simulink model "hopper_6dof_NED_v2_fluid_integration"  (R2026a)
settings: Solver=FixedStepAuto  StopTime=tgrid(end)  FixedStep=1e-3  RelTol=1e-5
InitFcn:
  | load('FuelPropsData.mat');
undefined symbols (not defined in the file): cg_init, dcg_dMfu_table, dcg_dMox_table, dI_dMfu_table, dI_dMox_table, ENGINE, engine_cg, engine_mass, fu_axial_damping_ratios, fu_lateral_damping_ratios, fu_mass_profile, fu_masses, fu_mdot_data, g, IN, K1flat, K2grid, MoI_init, mount_cg, OUT, ox_axial_damping_ratios, ox_lateral_damping_ratios, ox_mass_profile, ox_masses, ox_mdot_data, pressureLevels, r_leg, r_leg_1, r_leg_2, r_leg_3, r_leg_4, STRUCT, tank_r, TANKS, Target_Trajectory, tgrid, thrust_data, unom, uwndTable, VEH, vwndTable
libraries: fl_lib x43, nesl_utility x31, matrix_library x18, SimscapeFluids_lib x13, simulink x8, simulink_extras x7, slpidlib x7, dspindex x3, dspmtrx3 x3, sl_discontinuities x2, aerolibanim x1, commrandsrc3 x1
(part 1 of 7)
settings Model: Creator=asing  LastModifiedBy=asing
settings DebuggingCC: SignalInfNanChecking=warning
settings SimscapeCC: SimscapeNominalValues="[{\"value\":\"1\",\"unit\":\"A\"},{\"value\":\"1\",\"unit\":\"bar\"},{\"value\":\"1\",\"unit\":\"cm^2\"},{\"value\":\"1\",\"unit\":\"cm^3/s\"},{\"value\":\"1\",\"unit\":\"kJ/kg\"},{\"value\":\"1\",\"unit\":\"kW\"},{\"value\":\"1\",\"unit\":\"l\"},{\"value\":\"1\",\"unit\":\"N\"},{\"value\":\"1\",\"unit\":\"N*m\"},{\"value\":\"1\",\"unit\":\"V\"}]"  SimscapeLogType=none  SimscapeLogDataHistory=5000.0

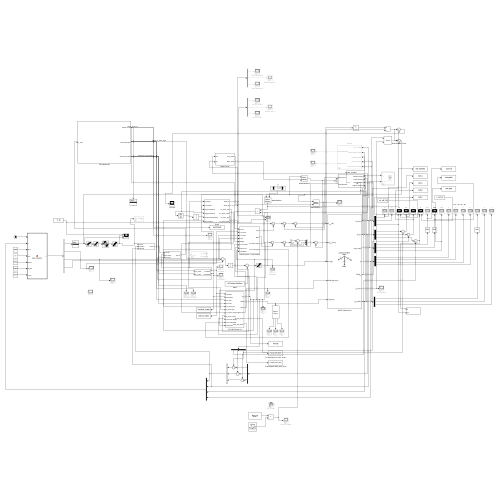
[thumbnail: Simulink's stored preview of the top-level diagram]
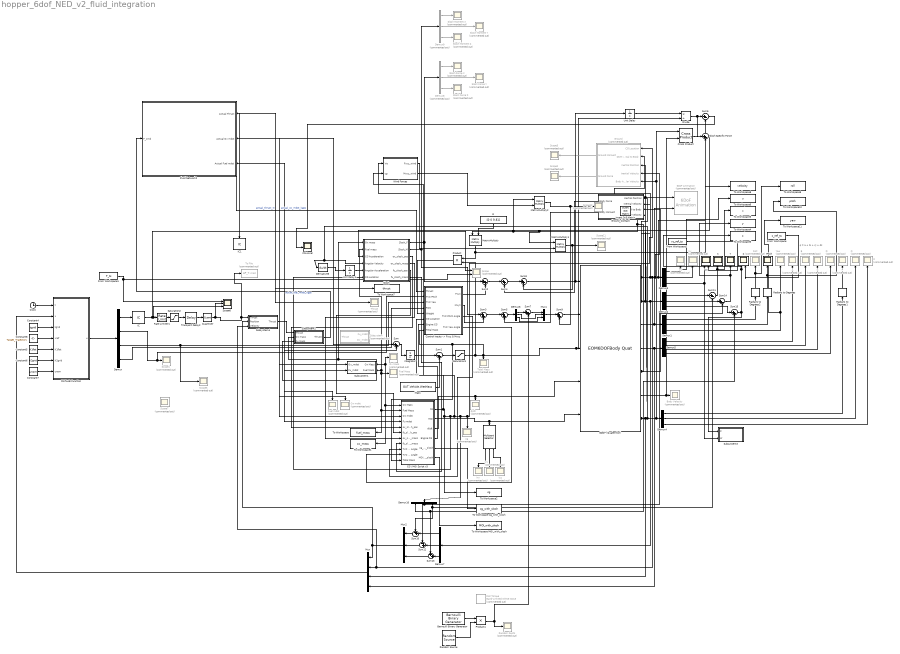
== system hopper_6dof_NED_v2_fluid_integration ==
  note: q = a + bi + cj + dk
  " " : dspindex/Multiport Selector  rowsOrCols=Rows  idxCellArray={1,2,3}  idxErrMode=Clip Index
      settings: LibrarySourceBlock=|
      | dsphdlsupportsigmgmt/Multiport
      | Selector
  6DOF (Quaternion) : EOM6DOFBodyQuat  mtype=Custom Variable  xme_0=[0 0 -cg_init]  eul_0=[0 pi/2 0]
  6DoF Animation : aerolibanim/6DoF Animation  Commented=on  u1=[0 200 -200 200 -100 5]  u2=0.1  u3=2  u4=[4000 0 -5000]  u5=Fly alongside  u6=[100 100 -50]  u7=10  u8=on
  A : Scope  Commented=on
      settings: ActiveDisplayYMinimum=-1  ActiveDisplayYMaximum=1  DataLoggingVariableName=ScopeData12
  B : Scope  Commented=on
      settings: ActiveDisplayYMinimum=-1  ActiveDisplayYMaximum=1  DataLoggingVariableName=ScopeData13
  Bernoulli Binary Generator : commrandsrc3/Bernoulli Binary Generator  ProbabilityOfZero=0.95  SeedSource=Parameter  Seed=0  SampleTime=0.1  SamplesPerFrame=1  OutputDataType=double  SimulateUsing=Interpreted execution
  Body Velocity : Scope  Commented=on
      settings: ActiveDisplayYMinimum=-9.910378836747423  ActiveDisplayYMaximum=88.214312640198585  DataLoggingVariableName=ScopeData29
  C : Scope  Commented=on
      settings: DataLoggingVariableName=ScopeData14
  CG / MOI Script v3 : Subsystem
  CG Accel : Scope
      settings: ActiveDisplayYMinimum=-11.407629776225166  ActiveDisplayYMaximum=3.5948297727236085  DataLoggingVariableName=ScopeData33
  Clock : Clock
  Constant4 : Constant  Value=tgrid
  Constant5 : Constant  Value=K1flat
  Constant6 : Constant  Value=K2grid
  Constant7 : Constant  Value=unom
  Constant8 : Constant  Value=Target_Trajectory
  "Control Inputs -> Fxyz & Mxyz" : Subsystem
  Cross Product : matrix_library/Cross Product
  D : Scope  Commented=on
      settings: DataLoggingVariableName=ScopeData15
  Demux : Demux
  Demux{1..4,6..7,10} (7 alike) : Demux  Outputs=3
  Demux5 : Demux
  Demux8 : Demux  Commented=on  Outputs=3
  Demux9 : Demux  Commented=on  Outputs=3
  Derivative3 : Derivative  CoefficientInTFapproximation=3
  Divide : Product  Inputs=*/
  Fluid Network2 : Subsystem
  From Workspace : FromWorkspace  VariableName=z_ref_ts
  From Workspace1 : FromWorkspace  VariableName=T_ts
  From Workspace2 : FromWorkspace  VariableName=vz_ref_ts
  Fuel Mass : Scope  Commented=on
      settings: ActiveDisplayYMinimum=7.5154679010584076  ActiveDisplayYMaximum=13.609392455437956  DataLoggingVariableName=ScopeData18
  Fuel mdot : Scope  Commented=on
      settings: ActiveDisplayYMinimum=-0.057229294241176995  ActiveDisplayYMaximum=0.515142758459371  DataLoggingVariableName=ScopeData20
  "Ground " : Subsystem  Commented=on
  Ground_Contact : Subsystem
  IC : InitialCondition  Value=VEH.mass.wet*g
  IC1 : InitialCondition  Value=VEH.mass.wet*g
  Integrator : Integrator
  Invert 3x3 Matrix : aerolibutil/Invert  3x3 Matrix
  Ixx : Scope  Commented=on
      settings: ActiveDisplayYMinimum=-1.2693672305907171  ActiveDisplayYMaximum=1.7662706804264152  DataLoggingVariableName=ScopeData21
  Iyy : Scope  Commented=on
      settings: ActiveDisplayYMinimum=-8.2381488489345962  ActiveDisplayYMaximum=64.485305245521346  DataLoggingVariableName=ScopeData26
  Izz : Scope  Commented=on
      settings: ActiveDisplayYMinimum=-8.2393172969859414  ActiveDisplayYMaximum=64.3796161087634  DataLoggingVariableName=ScopeData27
  MATLAB Function : MATLAB Function  TreatAsAtomicUnit=on
  Mass : Constant  Value=OUT.Vehicle.WetMass
  MatrixMultiply : Product  Multiplication=Matrix(*)
  MatrixMultiply1 : Product  Multiplication=Matrix(*)
  MatrixMultiply2 : Product  Multiplication=Matrix(*)
  Mux : Mux
  Mux1 : Mux  Inputs=3
  Mux2 : Mux  Inputs=3
  Ox Mass : Scope  Commented=on
      settings: ActiveDisplayYMinimum=9.14433500982005  ActiveDisplayYMaximum=16.761740554464438  DataLoggingVariableName=ScopeData17
  Ox mdot : Scope  Commented=on
      settings: ActiveDisplayYMinimum=-0.071536617800839461  ActiveDisplayYMaximum=0.64392844807434468  DataLoggingVariableName=ScopeData19
  P : Scope  Commented=on
      settings: ActiveDisplayYMinimum=-40.272034282628653  ActiveDisplayYMaximum=40.18271139614702  DataLoggingVariableName=ScopeData9
  Pitch : Scope
      settings: ActiveDisplayYMinimum=43.438097555335354  ActiveDisplayYMaximum=90.504604934017451  DataLoggingVariableName=ScopeData4
  Product : Product
  Product1 : Product
  Q : Scope  Commented=on
      settings: ActiveDisplayYMinimum=-0.03908687484475059  ActiveDisplayYMaximum=0.052615482319584864  DataLoggingVariableName=ScopeData10
  Quantizer : Quantizer  QuantizationInterval=IN.throttle_valve.resolution
  R : Scope  Commented=on
      settings: ActiveDisplayYMinimum=-0.0070860969112896514  ActiveDisplayYMaximum=0.0085398632976064828  DataLoggingVariableName=ScopeData11
  Radians to Degrees : simulink_extras/Transformations/Radians to Degrees
  Radians to Degrees1 : simulink_extras/Transformations/Radians to Degrees
  Radians to Degrees2 : simulink_extras/Transformations/Radians to Degrees
  Random Source : dspsrcs4/Random Source  SrcType=Gaussian  MinVal=0  MaxVal=1  MeanVal=0  VarVal=20  RepMode=Specify seed  rawSeed=1  IsInherit=off  SampTime=1  SampFrame=1  OutComplex=Real  DataType=double  SimulateUsing=Interpreted execution
  Random Gusts : Scope  Commented=on
      settings: ActiveDisplayYMinimum=-8.5897961122323956  ActiveDisplayYMaximum=9.8055336087823335  DataLoggingVariableName=ScopeData63
  Rate Limiter1 : RateLimiter  RisingSlewLimit=IN.throttle_valve.rate_limit  FallingSlewLimit=-IN.throttle_valve.rate_limit  SampleTimeMode=inherited
  Roll : Scope  Commented=on
      settings: ActiveDisplayYMinimum=-204.65947396986587  ActiveDisplayYMaximum=175.17097918939032  DataLoggingVariableName=ScopeData3
  Roll Torque : simulink/Sources/Band-Limited White Noise  Commented=on  Cov=5  Ts=1  seed=[23341]
  Saturation1 : Saturate  UpperLimit=OUT.Vehicle.WetMass  LowerLimit=OUT.Vehicle.DryMass
  Saturation2 : Saturate  UpperLimit=IN.propulsion.nominal_thrust * IN.propulsion.throttle_range(2)  LowerLimit=IN.propulsion.nominal_thrust * IN.propulsion.throttle_range(1)
  Scope : Scope  Commented=on  NumInputPorts=2
      settings: ActiveDisplayYMinimum=725.64918679567745  ActiveDisplayYMaximum=1423.3753088923004  DataLoggingVariableName=ScopeData52
  Scope{1..3,5,7,11..12} (7 alike) : Scope  Commented=on
      Scope1 settings: ActiveDisplayYMinimum=-0.00050229611394169284  ActiveDisplayYMaximum=0.0028458999197228797  DataLoggingVariableName=ScopeData53
      Scope11 settings: ActiveDisplayYMinimum=-1.725572479086533  ActiveDisplayYMaximum=0.1917302754540588  DataLoggingVariableName=ScopeData66
      Scope12 settings: ActiveDisplayYMinimum=-2.88543679656206  ActiveDisplayYMaximum=6.7910588943113428  DataLoggingVariableName=ScopeData67
      Scope2 settings: ActiveDisplayYMinimum=-8449.52436564975  ActiveDisplayYMaximum=76045.719290847759  DataLoggingVariableName=ScopeData49
      Scope3 settings: ActiveDisplayYMinimum=-903.54597657114152  ActiveDisplayYMaximum=89.720851920197276  DataLoggingVariableName=ScopeData51
      Scope5 settings: ActiveDisplayYMinimum=-0.0014807269526439936  ActiveDisplayYMaximum=0.00063209871075060983  DataLoggingVariableName=ScopeData57
      Scope7 settings: ActiveDisplayYMinimum=-9.3466701964128269  ActiveDisplayYMaximum=8.508922841651323  DataLoggingVariableName=ScopeData62
  Scope6 : Scope  NumInputPorts=3
      settings: ActiveDisplayYMinimum=-12632.794590273525  ActiveDisplayYMaximum=4410.2403285914115  DataLoggingVariableName=ScopeData59
  Slosh : Subsystem
  Slosh Force X : Scope  Commented=on
      settings: ActiveDisplayYMinimum=-23.703787957912279  ActiveDisplayYMaximum=30.843704332518367  DataLoggingVariableName=ScopeData32
  Slosh Force Y : Scope  Commented=on
      settings: ActiveDisplayYMinimum=-0.5552642189596475  ActiveDisplayYMaximum=0.52836332227705041  DataLoggingVariableName=ScopeData72
  Slosh Force Z : Scope  Commented=on
      settings: ActiveDisplayYMinimum=-0.4568274165323904  ActiveDisplayYMaximum=0.43197139726332079  DataLoggingVariableName=ScopeData73
  Slosh Moment X : Scope  Commented=on
      settings: ActiveDisplayYMinimum=-1  ActiveDisplayYMaximum=1  DataLoggingVariableName=ScopeData74
  Slosh Moment Y : Scope  Commented=on
      settings: ActiveDisplayYMinimum=-0.020821390947241118  ActiveDisplayYMaximum=0.019580844558623325  DataLoggingVariableName=ScopeData75
  Slosh Moment Z : Scope  Commented=on
      settings: ActiveDisplayYMinimum=-0.045380586631965543  ActiveDisplayYMaximum=0.048640802204673789  DataLoggingVariableName=ScopeData76
  Slosh Specific Force : Sum  Description=(F_total/m) - g_body = non-gravitational specific force at the CG; drives the slosh pendulums.  Inputs=|+-
  Subsystem : Subsystem  Commented=on
  Subsystem1 : Subsystem
  Subsystem2 : Subsystem
  Subsystem3 : Subsystem
  Subsystem4 : Subsystem
  Sum{,2..5,7..9,15} (9 alike) : Sum  Inputs=|++
  Sum1 : Sum  Inputs=|-+
  Sum10 : Sum  Inputs=-+|
  Sum11 : Sum  Inputs=|+-
  Sum12 : Sum  Inputs=-+|
  Sum13 : Sum  Inputs=++|
  Sum14 : Sum  Inputs=|+-
  Sum6 : Sum  Inputs=|+-
  Thrust : Scope  Commented=on
      settings: ActiveDisplayYMinimum=-212.49999999999994  ActiveDisplayYMaximum=1912.5  DataLoggingVariableName=ScopeData25
  To File : ToFile  Commented=on  Filename=AP_T.mat  SaveFormat=Timeseries
  To Workspace : ToWorkspace  VariableName=fuel_mass  SaveFormat=Timeseries  SampleTime=-1
  To Workspace MOI_with_slosh : ToWorkspace  VariableName=MOI_with_slosh  SaveFormat=Timeseries  SampleTime=-1
  To Workspace cg_with_slosh : ToWorkspace  VariableName=cg_with_slosh  SaveFormat=Timeseries  SampleTime=-1
  To Workspace1 : ToWorkspace  VariableName=ox_mass  SaveFormat=Timeseries  SampleTime=-1
  To Workspace10 : ToWorkspace  VariableName=pitch  SaveFormat=Timeseries  SampleTime=-1
  To Workspace11 : ToWorkspace  VariableName=yaw  SaveFormat=Timeseries  SampleTime=-1
  To Workspace2 : ToWorkspace  VariableName=cg  SaveFormat=Timeseries  SampleTime=-1
  To Workspace3 : ToWorkspace  VariableName=x  SaveFormat=Timeseries  SampleTime=-1
  To Workspace4 : ToWorkspace  VariableName=y  SaveFormat=Timeseries  SampleTime=-1
  To Workspace5 : ToWorkspace  VariableName=z  SaveFormat=Timeseries  SampleTime=-1
  To Workspace6 : ToWorkspace  VariableName=u  SaveFormat=Timeseries  SampleTime=-1
  To Workspace7 : ToWorkspace  VariableName=thrust  SaveFormat=Timeseries  SampleTime=-1
  To Workspace8 : ToWorkspace  VariableName=velocity  SaveFormat=Timeseries  SampleTime=-1
  To Workspace9 : ToWorkspace  VariableName=roll  SaveFormat=Timeseries  SampleTime=-1
  Total Mass : Scope  Commented=on
      settings: ActiveDisplayYMinimum=123.40007682459402  ActiveDisplayYMaximum=148.35554701948959  DataLoggingVariableName=ScopeData16
  Transport Delay2 : TransportDelay  DelayTime=IN.throttle_valve_latency
  Unit Delay : UnitDelay  SampleTime=-1
  Unit Delay1 : UnitDelay  SampleTime=-1
  Vx : Scope  Commented=on
      settings: ActiveDisplayYMinimum=-1.0568314607793221  ActiveDisplayYMaximum=0.63247821872235255  DataLoggingVariableName=ScopeData6
  Vy : Scope  Commented=on
      settings: ActiveDisplayYMinimum=-1  ActiveDisplayYMaximum=1  DataLoggingVariableName=ScopeData7
  Vz : Scope  NumInputPorts=2
      settings: ActiveDisplayYMinimum=-0.40844386646617703  ActiveDisplayYMaximum=1.313724578805866  DataLoggingVariableName=ScopeData8
  Wind Forces : Subsystem
  X : Scope
      settings: ActiveDisplayYMinimum=-0.57285266608571106  ActiveDisplayYMaximum=0.60376762362057124
  Y : Scope
      settings: ActiveDisplayYMinimum=-0.45246190447103363  ActiveDisplayYMaximum=0.388758387694069
  Yaw : Scope  Commented=on
      settings: ActiveDisplayYMinimum=-0.29772085399940185  ActiveDisplayYMaximum=2.6794861130407197  DataLoggingVariableName=ScopeData5
  Z : Scope  NumInputPorts=2
      settings: ActiveDisplayYMinimum=-0.11627941832016962  ActiveDisplayYMaximum=0.086760786687265876  DataLoggingVariableName=ScopeData2
  cg : Scope  Commented=on
      settings: ActiveDisplayYMinimum=-0.21955738430461946  ActiveDisplayYMaximum=1.426543136357856  DataLoggingVariableName=ScopeData23
  dI/dt : Scope  Commented=on
      settings: ActiveDisplayYMinimum=-0.25764178573017943  ActiveDisplayYMaximum=0.028626865081131041  DataLoggingVariableName=ScopeData22
  g : Constant  Value=[0 0 9.81]
  wires:
  6DOF (Quaternion)/2 -> "Ground "/3(Inertial Position), 6DoF Animation/1, Demux2/1, Demux7/1, Ground_Contact/1(Inertial Position)
  6DOF (Quaternion)/3 -> 6DoF Animation/2, Demux1/1
  Demux1/2 -> Radians to Degrees/1
  Demux3/1 -> To Workspace6/1, Vx/1
  Demux3/2 -> Vy/1
  6DOF (Quaternion)/4 -> Mux/4, Demux5/1
  Demux4/1 -> Radians to Degrees1/1
  Demux4/2 -> Q/1
  Demux4/3 -> R/1
  Demux5/1 -> A/1
  Demux5/2 -> B/1
  Demux5/3 -> C/1
  Demux5/4 -> D/1
  Demux3/3 -> Subsystem3/2(W), Vz/1
  Sum/1 -> Integrator/1
  Integrator/1 -> Sum1/1
  Mass/1 -> Sum1/2
  Sum1/1 -> Saturation1/1
  Saturation1/1 -> "Control Inputs -> Fxyz & Mxyz"/8(Total Mass), CG / MOI Script v3/11(Total Mass), Divide/2, 6DOF (Quaternion)/3, Total Mass/1, Product/2
  Subsystem1/2(Fuel Mass) -> Subsystem2/3(Fu mass), Slosh/2(Fuel mass), Fuel Mass/1, To Workspace/1, CG / MOI Script v3/2(Fuel Mass)
  CG / MOI Script v3/2(MOI) -> 6DOF (Quaternion)/5, " "/1
  CG / MOI Script v3/3(dI/dt) -> 6DOF (Quaternion)/4, dI/dt/1
  "Control Inputs -> Fxyz & Mxyz"/1(Fxyz) -> Sum2/2
  "Control Inputs -> Fxyz & Mxyz"/2(Mxyz) -> Sum3/2
  Subsystem1/1(Ox Mass) -> Subsystem2/2(Ox mass), Slosh/1(Ox mass), To Workspace1/1, CG / MOI Script v3/1(Ox Mass), Ox Mass/1
  6DOF (Quaternion)/6 -> Cross Product/2, Body Velocity/1
  MatrixMultiply/1 -> Product/1, Slosh Specific Force/2
  Invert 3x3 Matrix/1 -> "Ground "/2(DCM Inertial to Body)
  Sum2/1 -> Sum4/1
  Sum3/1 -> Sum5/1
  Cross Product/1 -> Sum6/2
  Divide/1 -> Sum6/1, Slosh Specific Force/1
  Sum6/1 -> CG Accel/1
  Unit Delay/1 -> Divide/1
  "Ground "/2(Ground Force) -> Scope2/1
  "Ground "/1(Ground Moment) -> Scope3/1
  Slosh/2(Slosh_M) -> Sum3/1, Demux9/1
  Slosh/1(Slosh_F) -> Demux8/1, Sum2/1
  Derivative3/1 -> Unit Delay1/1
  Product/1 -> "Control Inputs -> Fxyz & Mxyz"/5(Weight)
  Demux1/1 -> Radians to Degrees2/1
  Demux1/3 -> Yaw/1, To Workspace11/1
  g/1 -> MatrixMultiply/2
  Clock/1 -> MATLAB Function/1(t)
  Constant7/1 -> MATLAB Function/7(unom)
  Constant5/1 -> MATLAB Function/5(K1flat)
  Mux/1 -> MATLAB Function/2(x)
  Constant8/1 -> MATLAB Function/4(xref)
  Constant4/1 -> MATLAB Function/3(tgrid)
  Constant6/1 -> MATLAB Function/6(K2grid)
  Rate Limiter1/1 -> Saturation2/1
  MATLAB Function/1(u) -> Demux/1
  Demux/2 -> "Control Inputs -> Fxyz & Mxyz"/2(TVC Pitch), Scope1/1
  Demux/3 -> "Control Inputs -> Fxyz & Mxyz"/3(TVC Yaw), Scope5/1
  Demux/1 -> IC/1
  Transport Delay2/1 -> Quantizer/1
  From Workspace1/1 -> Scope6/1, Scope/2
  IC/1 -> Scope/1, Scope6/3, Rate Limiter1/1
  From Workspace2/1 -> Vz/2
  Sum7/1 -> Mux1/1
  Demux6/1 -> Sum7/1
  Demux6/2 -> Mux1/2
  Demux6/3 -> Mux1/3
  Sum5/1 -> Demux6/1
  Wind Forces/2(Mxyz_wind) -> MatrixMultiply2/2
  6DOF (Quaternion)/1 -> Wind Forces/1(Ve), Subsystem4/3(Velocity), Mux/2, "Ground "/4(Inertial Velocity), To Workspace8/1, Demux3/1, Ground_Contact/2(Inertial Velocity)
  Sum8/1 -> Unit Delay/1, 6DOF (Quaternion)/1
  Sum4/1 -> Sum8/1
  Mux1/1 -> Sum9/1
  Sum9/1 -> 6DOF (Quaternion)/2
  6DOF (Quaternion)/5 -> MatrixMultiply1/1, MatrixMultiply2/1, MatrixMultiply/1, Invert 3x3 Matrix/1, Ground_Contact/3(Inertial to Body)
  Wind Forces/1(Fxyz_wind) -> MatrixMultiply1/2
  MatrixMultiply1/1 -> Sum8/2, Scope11/1
  MatrixMultiply2/1 -> Sum9/2, Scope12/1
  Mux2/1 -> Mux/1, Subsystem4/2(Position)
  CG / MOI Script v3/1(cg) -> Wind Forces/2(cg), To Workspace2/1, Slosh/6(CG Location), Demux10/1, "Ground "/1(CG Location), cg/1, "Control Inputs -> Fxyz & Mxyz"/6(CG Location)
  Demux8/1 -> Slosh Force X/1
  Demux8/2 -> Slosh Force Y/1
  Demux8/3 -> Slosh Force Z/1
  Demux9/1 -> Slosh Moment X/1
  Demux9/2 -> Slosh Moment Y/1
  Demux9/3 -> Slosh Moment Z/1
  Subsystem4/1("Thrust ") -> Subsystem2/1(Thrust)
  Saturation2/1 -> Transport Delay2/1
  Quantizer/1 -> Scope6/2, Subsystem4/1(Thrust), To File/1
  6DOF (Quaternion)/7 -> Mux/3, "Ground "/5(Body Angular Velocity), Cross Product/1, Demux4/1, Derivative3/1, Slosh/4(Angular Velocity), Ground_Contact/4(Angular Velocity)
  Demux7/1 -> Sum10/2
  Sum10/1 -> Mux2/1
  Sum12/1 -> Mux2/2
  Demux7/2 -> Sum12/2
  Demux7/3 -> Sum13/2
  Sum13/1 -> Mux2/3
  Demux10/2 -> Sum14/2, Sum12/1
  Demux10/3 -> Sum11/2, Sum10/1
  Demux10/1 -> Sum15/2, Sum13/1
  Demux2/1 -> Sum11/1
  Sum11/1 -> To Workspace3/1, X/1
  Demux2/2 -> Sum14/1
  Sum14/1 -> To Workspace4/1, Y/1
  Demux2/3 -> Sum15/1
  Slosh/3(ox_slosh_pos) -> CG / MOI Script v3/5(ox_slosh_pos)
  Slosh/4(ox_slosh_mass) -> CG / MOI Script v3/7(ox_slosh_mass)
  Slosh/5(fu_slosh_pos) -> CG / MOI Script v3/6(fu_slosh_pos)
  Slosh/6(fu_slosh_mass) -> CG / MOI Script v3/8(fu_slosh_mass)
  "Control Inputs -> Fxyz & Mxyz"/3(TVC Pitch Angle) -> CG / MOI Script v3/9(TVC Pitch Angle)
  "Control Inputs -> Fxyz & Mxyz"/4(TVC Yaw Angle) -> CG / MOI Script v3/10(TVC Yaw Angle)
  CG / MOI Script v3/4(Engine CG) -> "Control Inputs -> Fxyz & Mxyz"/7(Engine CG)
  " "/1 -> Ixx/1
  " "/2 -> Iyy/1
  " "/3 -> Izz/1
  Unit Delay1/1 -> Slosh/5(Angular Acceleration)
  Demux/4 -> "Control Inputs -> Fxyz & Mxyz"/4("RCS ")
  Radians to Degrees/1 -> To Workspace10/1, Pitch/1
  Sum15/1 -> To Workspace5/1, Z/1, Subsystem3/1(Z)
  From Workspace/1 -> Z/2
  Bernoulli Binary Generator/1 -> Product1/1
  Random Source/1 -> Product1/2
  Product1/1 -> Sum7/2, Random Gusts/1
  Radians to Degrees1/1 -> P/1
  Radians to Degrees2/1 -> To Workspace9/1, Roll/1
  Slosh Specific Force/1 -> Slosh/3(CG Acceleration)
  CG / MOI Script v3/5(cg_with_slosh) -> To Workspace cg_with_slosh/1
  CG / MOI Script v3/6(MOI_with_slosh) -> To Workspace MOI_with_slosh/1
  Subsystem2/1("Thrust ") -> Fluid Network2/1(F_cmd)
  Fluid Network2/1(Actual Thrust) -> IC1/1, "Control Inputs -> Fxyz & Mxyz"/1("Thrust "), To Workspace7/1, Thrust/1  "actual_thrust_N"
  Fluid Network2/2(Actual Ox mdot) -> Sum/1, Subsystem1/1(Ox_mdot), CG / MOI Script v3/3(Ox mdot), Ox mdot/1  "actual_ox_mdot_kgps"
  Fluid Network2/3(Actual Fuel mdot) -> Sum/2, Subsystem1/2(Fu_mdot), Fuel mdot/1, CG / MOI Script v3/4(Fu mdot)  "actual_fuel_mdot_kgps"
  Ground_Contact/1(Body Force) -> Sum4/2
  Ground_Contact/2(Body Moment) -> Sum5/2

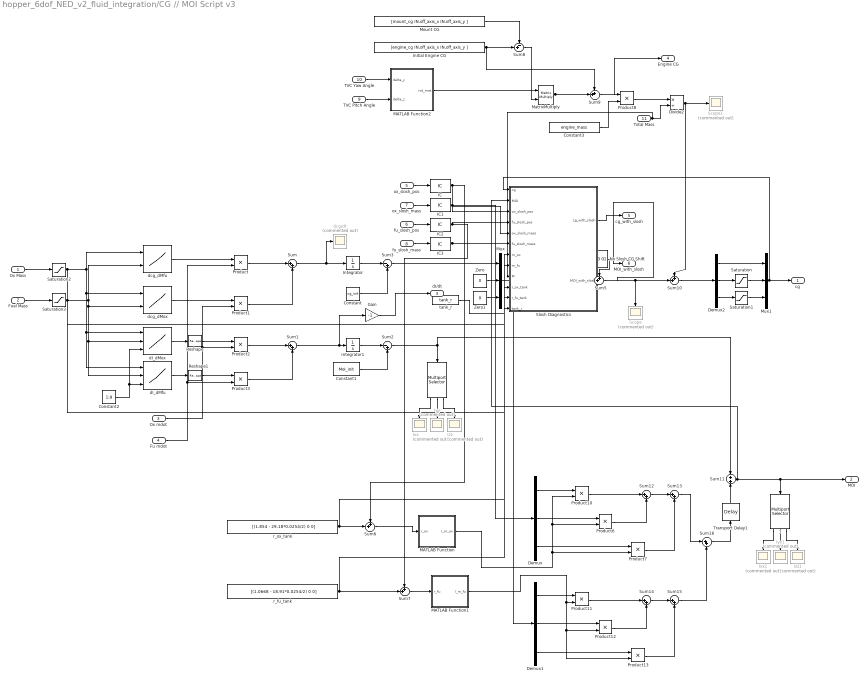
== system hopper_6dof_NED_v2_fluid_integration/CG // MOI Script v3 ==
  Ox Mass : Inport
  Fuel Mass : Inport  Port=2
  Ox mdot : Inport  Port=3
  Fu mdot : Inport  Port=4
  ox_slosh_pos : Inport  Port=5
  fu_slosh_pos : Inport  Port=6
  ox_slosh_mass : Inport  Port=7
  fu_slosh_mass : Inport  Port=8
  TVC Pitch Angle : Inport  Port=9
  TVC Yaw Angle : Inport  Port=10
  Total Mass : Inport  Port=11
  " " : dspindex/Multiport Selector  rowsOrCols=Rows  idxCellArray={1,2,3}  idxErrMode=Clip Index
      settings: LibrarySourceBlock=|
      | dsphdlsupportsigmgmt/Multiport
      | Selector
  " 1" : dspindex/Multiport Selector  rowsOrCols=Rows  idxCellArray={1,2,3}  idxErrMode=Clip Index
      settings: LibrarySourceBlock=|
      | dsphdlsupportsigmgmt/Multiport
      | Selector
  Constant : Constant  Value=cg_init
  Constant1 : Constant  Value=MoI_init
  Constant2 : Constant  Value=1:9
  Constant3 : Constant  Value=engine_mass
  Demux : Demux  Outputs=3
  Demux1 : Demux  Outputs=3
  Demux2 : Demux  Outputs=3
  Divide2 : Product  Inputs=*/
  Gain : Gain  Gain=-1
  IC{,1..3} (4 alike) : InitialCondition  Value=[0 0 0]
  Initial Engine CG : Constant  Value=[engine_cg IN.off_axis_x IN.off_axis_y ]
  Integrator : Integrator
  Integrator1 : Integrator
  Ixx : Scope  Commented=on
      settings: ActiveDisplayYMinimum=-3.1515489726992576  ActiveDisplayYMaximum=1.474087451117061  DataLoggingVariableName=ScopeData19
  Ixx1 : Scope  Commented=on
      settings: ActiveDisplayYMinimum=-1.0489589814194713  ActiveDisplayYMaximum=1.2999685130860112  DataLoggingVariableName=ScopeData64
  Iyy : Scope  Commented=on
      settings: ActiveDisplayYMinimum=30.163212884427733  ActiveDisplayYMaximum=49.780093450314517  DataLoggingVariableName=ScopeData20
  Iyy1 : Scope  Commented=on
      settings: ActiveDisplayYMinimum=-7.7835032784132139  ActiveDisplayYMaximum=64.56514685530945  DataLoggingVariableName=ScopeData65
  Izz : Scope  Commented=on
      settings: ActiveDisplayYMinimum=-2.8210574648941242  ActiveDisplayYMaximum=25.389517184047122  DataLoggingVariableName=ScopeData22
  Izz1 : Scope  Commented=on
      settings: ActiveDisplayYMinimum=-8.0012534921806147  ActiveDisplayYMaximum=64.52262360939288  DataLoggingVariableName=ScopeData68
  MATLAB Function : MATLAB Function  TreatAsAtomicUnit=on
  MATLAB Function1 : MATLAB Function  TreatAsAtomicUnit=on
  MATLAB Function2 : MATLAB Function  TreatAsAtomicUnit=on
  MatrixMultiply : Product  Multiplication=Matrix(*)
  Mount CG : Constant  Value=[mount_cg IN.off_axis_x IN.off_axis_y ]
  Mux : Mux  Inputs=3
  Mux1 : Mux  Inputs=3
  No Slosh CG Shift : Constant  Description=Slosh mass offset now enters as a moment in Slosh/Ox|Fu Slosh Offset Moment.  Value=[0 0 0]
  Product{,1..3,6..7,10..13} (10 alike) : Product
  Product8 : Product  Description=Engine moment change from gimballing: m_engine * displacement. cg_init already contains the engine at its nominal position.
  Reshape : Reshape  OutputDimensionality=Customize  OutputDimensions=[3,3]
  Reshape1 : Reshape  OutputDimensionality=Customize  OutputDimensions=[3,3]
  Saturation : Saturate  UpperLimit=tank_r  LowerLimit=-tank_r
  Saturation1 : Saturate  UpperLimit=tank_r  LowerLimit=-tank_r
  Saturation2 : Saturate  UpperLimit=inf  LowerLimit=0.01
  Saturation3 : Saturate  UpperLimit=inf  LowerLimit=0.01
  Scope : Scope  Commented=on
      settings: ActiveDisplayYMinimum=-1  ActiveDisplayYMaximum=1  DataLoggingVariableName=ScopeData18
  Scope1 : Scope  Commented=on
      settings: ActiveDisplayYMinimum=-0.011780085539767782  ActiveDisplayYMaximum=0.093584740104547162  DataLoggingVariableName=ScopeData77
  Slosh Diagnostics : MATLAB Function  TreatAsAtomicUnit=on
  Sum{,1,12..16} (7 alike) : Sum  Inputs=|++
  Sum{5..7,10} (4 alike) : Sum  Inputs=++|
  Sum11 : Sum  Inputs=+|+
  Sum2 : Sum  Inputs=|-+
  Sum3 : Sum  Inputs=|-+
  Sum8 : Sum  Inputs=-+|
  Sum9 : Sum  Description=Gimballed engine CG = engine CG + small-angle rotation of (engine - mount) about the mount. Lies on the thrust line.  Inputs=++|
  Transport Delay1 : TransportDelay  DelayTime=0.01
  Zero : Constant  Value=0  OutDataTypeStr=Inherit: Inherit via back propagation
  Zero1 : Constant  Value=0  OutDataTypeStr=Inherit: Inherit via back propagation
  dI_dMfu : Lookup_n-D  NumberOfTableDimensions=3  BreakpointsForDimension1=ox_masses  BreakpointsForDimension2=fu_masses  BreakpointsForDimension3=1:9  Table=dI_dMfu_table  InternalRulePriority=Speed  RndMeth=Simplest
      settings: InputPortMap=u0,u1,u2
  dI_dMox : Lookup_n-D  NumberOfTableDimensions=3  BreakpointsForDimension1=ox_masses  BreakpointsForDimension2=fu_masses  BreakpointsForDimension3=1:9  Table=dI_dMox_table  InternalRulePriority=Speed  RndMeth=Simplest
      settings: InputPortMap=u0,u1,u2
  dcg/dt : Scope  Commented=on
      settings: ActiveDisplayYMinimum=-0.00024176262833681272  ActiveDisplayYMaximum=0.0021761772093484262  DataLoggingVariableName=ScopeData41
  dcg_dMfu : Lookup_n-D  BreakpointsForDimension1=ox_masses  BreakpointsForDimension2=fu_masses  BreakpointsForDimension3=[5, 7]  Table=dcg_dMfu_table  InternalRulePriority=Speed  RndMeth=Simplest
      settings: InputPortMap=u0,u1
  dcg_dMox : Lookup_n-D  BreakpointsForDimension1=ox_masses  BreakpointsForDimension2=fu_masses  BreakpointsForDimension3=[5, 7]  Table=dcg_dMox_table  InternalRulePriority=Speed  RndMeth=Simplest
      settings: InputPortMap=u0,u1
  r_fu_tank : Constant  Value=[(1.0668 - 18.91*0.0254/2) 0 0]
  r_ox_tank : Constant  Value=[(1.854 - 29.18*0.0254/2) 0 0]
  tank_r : Constant  Value=tank_r
  cg : Outport
  MOI : Outport  Port=2
  dI/dt : Outport  Port=3
  Engine CG : Outport  Port=4
  cg_with_slosh : Outport  Port=5
  MOI_with_slosh : Outport  Port=6
  wires:
  Ox Mass/1 -> Saturation2/1
  Fuel Mass/1 -> Saturation3/1
  dcg_dMfu/1 -> Product/1
  Ox mdot/1 -> Product2/2, Product1/2
  dcg_dMox/1 -> Product1/1
  Fu mdot/1 -> Product3/2, Product/2
  dI_dMox/1 -> Reshape/1
  dI_dMfu/1 -> Reshape1/1
  Product/1 -> Sum/1
  Product1/1 -> Sum/2
  Product2/1 -> Sum1/1
  Product3/1 -> Sum1/2
  Sum/1 -> dcg/dt/1, Integrator/1
  Integrator/1 -> Sum3/1
  Constant/1 -> Sum3/2
  Sum1/1 -> Gain/1, Integrator1/1
  Integrator1/1 -> Sum2/1
  Constant1/1 -> Sum2/2
  Reshape/1 -> Product2/1
  Reshape1/1 -> Product3/1
  Constant2/1 -> dI_dMfu/3, dI_dMox/3
  " "/2 -> Iyy/1
  " "/1 -> Ixx/1
  " "/3 -> Izz/1
  Sum2/1 -> Sum11/1, " "/1
  Gain/1 -> dI/dt/1
  Sum3/1 -> Mux/1
  Zero/1 -> Mux/2
  Zero1/1 -> Mux/3
  Mux/1 -> Sum5/2
  ox_slosh_pos/1 -> IC/1
  ox_slosh_mass/1 -> IC1/1
  fu_slosh_pos/1 -> IC2/1
  fu_slosh_mass/1 -> IC3/1
  IC/1 -> Sum6/1, Slosh Diagnostics/3(ox_slosh_pos)
  IC2/1 -> Sum7/1, Slosh Diagnostics/4(fu_slosh_pos)
  IC3/1 -> Demux1/1, Slosh Diagnostics/6(fu_slosh_mass)
  Sum5/1 -> Sum10/2, Scope/1
  r_ox_tank/1 -> Sum6/2, Slosh Diagnostics/10(r_ox_tank)
  r_fu_tank/1 -> Sum7/2, Slosh Diagnostics/11(r_fu_tank)
  " 1"/1 -> Ixx1/1
  " 1"/2 -> Iyy1/1
  " 1"/3 -> Izz1/1
  Sum11/1 -> MOI/1, " 1"/1, Slosh Diagnostics/2(MOI)
  IC1/1 -> Demux/1, Slosh Diagnostics/5(ox_slosh_mass)
  Demux/1 -> Product10/1
  Demux/2 -> Product6/1
  Demux/3 -> Product7/1
  Product10/1 -> Sum12/1
  Product6/1 -> Sum12/2
  Sum12/1 -> Sum13/1
  Product7/1 -> Sum13/2
  Sum14/1 -> Sum15/1
  Demux1/2 -> Product12/1
  Product12/1 -> Sum14/2
  Demux1/3 -> Product13/1
  Product13/1 -> Sum15/2
  Product11/1 -> Sum14/1
  Demux1/1 -> Product11/1
  Sum13/1 -> Sum16/1
  Sum15/1 -> Sum16/2
  Sum16/1 -> Transport Delay1/1
  Sum6/1 -> MATLAB Function/1(r_ox)
  Sum7/1 -> MATLAB Function1/1(r_fu)
  MATLAB Function/1(I_m_ox) -> Product7/2, Product6/2, Product10/2
  MATLAB Function1/1(I_m_fu) -> Product13/2, Product12/2, Product11/2
  Transport Delay1/1 -> Sum11/2
  Demux2/2 -> Saturation/1
  Demux2/1 -> Mux1/1
  Demux2/3 -> Saturation1/1
  Saturation/1 -> Mux1/2
  Saturation1/1 -> Mux1/3
  Mux1/1 -> cg/1, Slosh Diagnostics/1(cg)
  TVC Pitch Angle/1 -> MATLAB Function2/2(delta_z)
  TVC Yaw Angle/1 -> MATLAB Function2/1(delta_y)
  Initial Engine CG/1 -> Sum8/2, Sum9/1
  Mount CG/1 -> Sum8/1
  MATLAB Function2/1(rot_mat) -> MatrixMultiply/1
  Sum8/1 -> MatrixMultiply/2
  MatrixMultiply/1 -> Sum9/2, Product8/1
  Sum9/1 -> Engine CG/1
  Constant3/1 -> Product8/2
  Product8/1 -> Divide2/1
  Total Mass/1 -> Divide2/2, Slosh Diagnostics/9(M)
  Divide2/1 -> Sum10/1, Scope1/1
  Sum10/1 -> Demux2/1
  Saturation2/1 -> dI_dMfu/1, dI_dMox/1, dcg_dMox/1, dcg_dMfu/1, Slosh Diagnostics/7(m_ox)
  Saturation3/1 -> dI_dMfu/2, dI_dMox/2, dcg_dMox/2, dcg_dMfu/2, Slosh Diagnostics/8(m_fu)
  No Slosh CG Shift/1 -> Sum5/1
  tank_r/1 -> Slosh Diagnostics/12(tank_r)
  Slosh Diagnostics/1(cg_with_slosh) -> cg_with_slosh/1
  Slosh Diagnostics/2(MOI_with_slosh) -> MOI_with_slosh/1

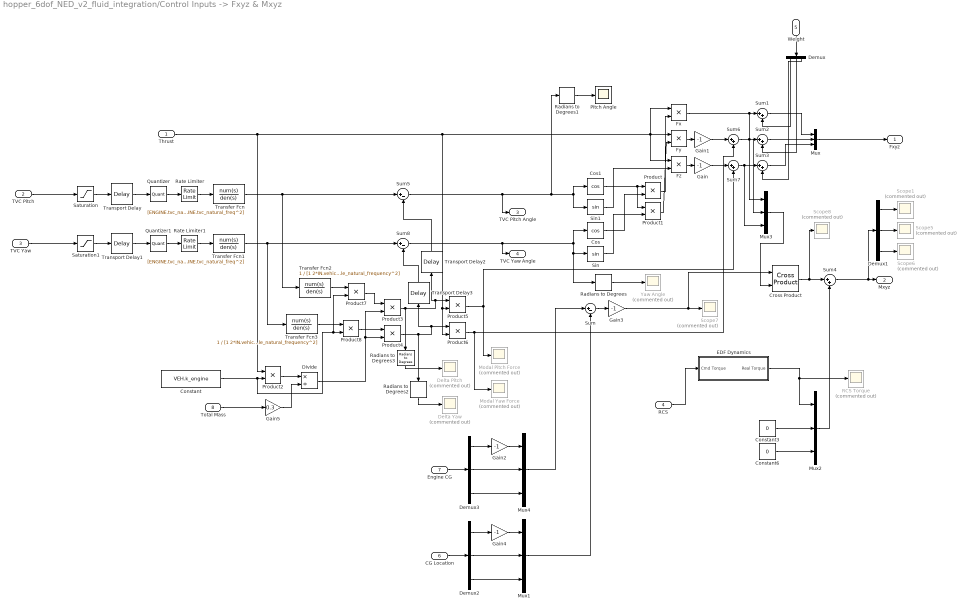
== system hopper_6dof_NED_v2_fluid_integration/Control Inputs -> Fxyz & Mxyz ==
  "Thrust " : Inport
  TVC Pitch : Inport  Port=2
  TVC Yaw : Inport  Port=3
  "RCS " : Inport  Port=4
  Weight : Inport  Port=5
  CG Location : Inport  Port=6
  Engine CG : Inport  Port=7
  Total Mass : Inport  Port=8
  Constant : Constant  Value=VEH.k_engine
  Constant3 : Constant  Value=0
  Constant6 : Constant  Value=0
  Cos : Trigonometry  Operator=cos
  Cos1 : Trigonometry  Operator=cos
  Cross Product : matrix_library/Cross Product
  Delta Pitch : Scope  Commented=on
      settings: ActiveDisplayYMinimum=-0.0038016775387335047  ActiveDisplayYMaximum=0.0038576393364572227  DataLoggingVariableName=ScopeData83
  Delta Yaw : Scope  Commented=on
      settings: ActiveDisplayYMinimum=-0.0018754271280055322  ActiveDisplayYMaximum=0.0029155281667496203  DataLoggingVariableName=ScopeData84
  Demux{,1..3} (4 alike) : Demux  Outputs=3
  Divide : Product  Inputs=*/
  EDF Dynamics : Subsystem
  Fx : Product
  Fy : Product
  Fz : Product
  Gain{,1..4} (5 alike) : Gain  Gain=-1
  Gain5 : Gain  Gain=0.3
  Modal Pitch Force : Scope  Commented=on
      settings: ActiveDisplayYMinimum=-0.088739631277941974  ActiveDisplayYMaximum=0.086025104693778914  DataLoggingVariableName=ScopeData78
  Modal Yaw Force : Scope  Commented=on
      settings: ActiveDisplayYMinimum=-0.017420268895536287  ActiveDisplayYMaximum=0.028077380315148965  DataLoggingVariableName=ScopeData79
  Mux{,1..4} (5 alike) : Mux  Inputs=3
  Pitch Angle : Scope
      settings: ActiveDisplayYMinimum=-10.903439073445846  ActiveDisplayYMaximum=7.4616563198748231  DataLoggingVariableName=ScopeData71
  Product{,1..8} (9 alike) : Product
  Quantizer : Quantizer  QuantizationInterval=IN.tvc.resolution
  Quantizer1 : Quantizer  QuantizationInterval=IN.tvc.resolution
  RCS Torque : Scope  Commented=on
      settings: ActiveDisplayYMinimum=-8.021209014289818  ActiveDisplayYMaximum=10.60123996530198  DataLoggingVariableName=ScopeData47
  Radians to Degrees{,1..3} (4 alike) : simulink_extras/Transformations/Radians to Degrees
  Rate Limiter : RateLimiter  RisingSlewLimit=IN.tvc.max_gimbal_rate  FallingSlewLimit=-IN.tvc.max_gimbal_rate  SampleTimeMode=inherited
  Rate Limiter1 : RateLimiter  RisingSlewLimit=IN.tvc.max_gimbal_rate  FallingSlewLimit=-IN.tvc.max_gimbal_rate  SampleTimeMode=inherited
  Saturation : Saturate  UpperLimit=IN.tvc.max_gimbal_angle  LowerLimit=-IN.tvc.max_gimbal_angle
  Saturation1 : Saturate  UpperLimit=IN.tvc.max_gimbal_angle  LowerLimit=-IN.tvc.max_gimbal_angle  LinearizeAsGain=off
  Scope{1,5..8} (5 alike) : Scope  Commented=on
      Scope1 settings: ActiveDisplayYMinimum=0.090000000000000011  ActiveDisplayYMaximum=0.11  DataLoggingVariableName=ScopeData50
      Scope5 settings: ActiveDisplayYMinimum=-1  ActiveDisplayYMaximum=1  DataLoggingVariableName=ScopeData54
      Scope6 settings: ActiveDisplayYMinimum=-1  ActiveDisplayYMaximum=1  DataLoggingVariableName=ScopeData55
      Scope7 settings: ActiveDisplayYMinimum=-1.008334185713273  ActiveDisplayYMaximum=-0.924758879501166  DataLoggingVariableName=ScopeData56
      Scope8 settings: ActiveDisplayYMinimum=-1  ActiveDisplayYMaximum=1  DataLoggingVariableName=ScopeData60
  Sin : Trigonometry
  Sin1 : Trigonometry
  Sum : Sum  Inputs=|+-
  Sum{1..4,6..7} (6 alike) : Sum  Inputs=|++
  Sum5 : Sum  Inputs=|+-
  Sum8 : Sum  Inputs=|+-
  Transfer Fcn : TransferFcn  Numerator=[ENGINE.tvc_natural_freq^2]  Denominator=[1 2*IN.tvc.damping_ratio*ENGINE.tvc_natural_freq ENGINE.tvc_natural_freq^2]
  Transfer Fcn1 : TransferFcn  Numerator=[ENGINE.tvc_natural_freq^2]  Denominator=[1 2*IN.tvc.damping_ratio*ENGINE.tvc_natural_freq ENGINE.tvc_natural_freq^2]
  Transfer Fcn2 : TransferFcn  Numerator=1  Denominator=[1 2*IN.vehicle_damping_ratio*IN.vehicle_natural_frequency IN.vehicle_natural_frequency^2]
  Transfer Fcn3 : TransferFcn  Numerator=1  Denominator=[1 2*IN.vehicle_damping_ratio*IN.vehicle_natural_frequency IN.vehicle_natural_frequency^2]
  Transport Delay : TransportDelay  DelayTime=IN.tvc.actuator_latency
  Transport Delay1 : TransportDelay  DelayTime=IN.tvc.actuator_latency
  Transport Delay2 : TransportDelay  DelayTime=0.01
  Transport Delay3 : TransportDelay  DelayTime=0.01
  Yaw Angle : Scope  Commented=on
      settings: ActiveDisplayYMinimum=-1.8231379337691429  ActiveDisplayYMaximum=5.2718467554145434  DataLoggingVariableName=ScopeData70
  Fxyz : Outport
  Mxyz : Outport  Port=2
  TVC Pitch Angle : Outport  Port=3
  TVC Yaw Angle : Outport  Port=4
  wires:
  Cos1/1 -> Product1/1, Product/1
  Cos/1 -> Product/2
  Product/1 -> Fx/2
  "Thrust "/1 -> Product2/1, Product6/2, Product5/2, Fx/1, Fy/1, Fz/1
  Mux/1 -> Fxyz/1
  Sum1/1 -> Mux/1
  Weight/1 -> Demux/1
  Fy/1 -> Gain1/1
  Sum2/1 -> Mux/2
  Fz/1 -> Gain/1
  Demux/2 -> Sum2/2
  Mux1/1 -> Sum/2
  Sum/1 -> Gain3/1
  Cross Product/1 -> Scope8/1, Sum4/1
  Constant3/1 -> Mux2/2
  Mux2/1 -> Sum4/2
  Saturation/1 -> Transport Delay/1
  Saturation1/1 -> Transport Delay1/1
  Sum4/1 -> Demux1/1, Mxyz/1
  Demux1/1 -> Scope1/1
  Demux1/2 -> Scope5/1
  Demux1/3 -> Scope6/1
  Product1/1 -> Fy/2
  Sin/1 -> Product1/2
  Sin1/1 -> Fz/2
  Gain3/1 -> Cross Product/1, Scope7/1
  Sum3/1 -> Mux/3
  Mux3/1 -> Cross Product/2
  Constant6/1 -> Mux2/3
  Demux/1 -> Sum1/2
  Demux/3 -> Sum3/2
  Transport Delay/1 -> Quantizer/1
  Transport Delay1/1 -> Quantizer1/1
  Radians to Degrees/1 -> Yaw Angle/1
  Radians to Degrees1/1 -> Pitch Angle/1
  "RCS "/1 -> EDF Dynamics/1(Cmd Torque)
  Quantizer/1 -> Rate Limiter/1
  Quantizer1/1 -> Rate Limiter1/1
  Rate Limiter/1 -> Transfer Fcn/1
  Rate Limiter1/1 -> Transfer Fcn1/1
  TVC Pitch/1 -> Saturation/1
  TVC Yaw/1 -> Saturation1/1
  Transfer Fcn/1 -> Sum5/1, Transfer Fcn2/1
  Transfer Fcn1/1 -> Sum8/1, Transfer Fcn3/1
  Demux2/3 -> Mux1/3
  CG Location/1 -> Demux2/1
  Demux2/2 -> Mux1/2
  Demux2/1 -> Gain4/1
  Gain4/1 -> Mux1/1
  Gain2/1 -> Mux4/1
  Demux3/1 -> Gain2/1
  Demux3/2 -> Mux4/2
  Demux3/3 -> Mux4/3
  Engine CG/1 -> Demux3/1
  Mux4/1 -> Sum/1
  Total Mass/1 -> Gain5/1
  Product2/1 -> Divide/1
  Gain5/1 -> Divide/2
  Constant/1 -> Product7/2, Product8/2, Product2/2
  Divide/1 -> Product3/2, Product4/2
  Product3/1 -> Transport Delay2/1, Product5/1, Radians to Degrees3/1
  Product4/1 -> Radians to Degrees2/1, Transport Delay3/1, Product6/1
  Fx/1 -> Mux3/1, Sum1/1
  Gain1/1 -> Sum6/1
  Sum6/1 -> Mux3/2, Sum2/1
  Gain/1 -> Sum7/1
  Sum7/1 -> Sum3/1, Mux3/3
  Product5/1 -> Sum7/2, Modal Pitch Force/1
  Product6/1 -> Sum6/2, Modal Yaw Force/1
  Sum5/1 -> TVC Pitch Angle/1, Radians to Degrees1/1, Sin1/1, Cos1/1
  Sum8/1 -> TVC Yaw Angle/1, Sin/1, Radians to Degrees/1, Cos/1
  Radians to Degrees2/1 -> Delta Yaw/1
  Radians to Degrees3/1 -> Delta Pitch/1
  Transport Delay3/1 -> Sum8/2
  Transport Delay2/1 -> Sum5/2
  Transfer Fcn2/1 -> Product7/1
  Product7/1 -> Product3/1
  Transfer Fcn3/1 -> Product8/1
  Product8/1 -> Product4/1
  EDF Dynamics/1("Real Torque ") -> Mux2/1, RCS Torque/1
